simulink model "hysteresis_pam3_compare"  (R2022a)
settings: Solver=FixedStepDiscrete  StartTime=0  StopTime=simple_stop_time  FixedStep=simple_ts  RelTol=1e-3
undefined symbols (not defined in the file): simple_cfg, simple_ts
Description:
  | Structural preview, not MATLAB-saved or Simulink-tested. Run START_SIMULINK_COMPARE to rebuild natively and validate.
settings SolverCC: AlgebraicLoopSolver=TrustRegion
settings DataIOCC: SaveFormat=Array  SaveOutput=off  SignalLogging=off  TimeSaveName=simple_time
settings OptimizationCC: LifeSpan=inf
settings DebuggingCC: UnconnectedInputMsg=warning  UnconnectedOutputMsg=warning  UnconnectedLineMsg=warning  SFMachineParentedDataDiag=warning  ArithmeticOperatorsInVariantConditions=warning
settings SFSimCC: SimUseLocalCustomCode=off  CustomCodeUndefinedFunction=UseInterfaceOnly
settings RTWCC: RTWUseLocalCustomCode=off  DLArmComputeVersion=19.05
settings CodeAppCC: StateflowObjectComments=on

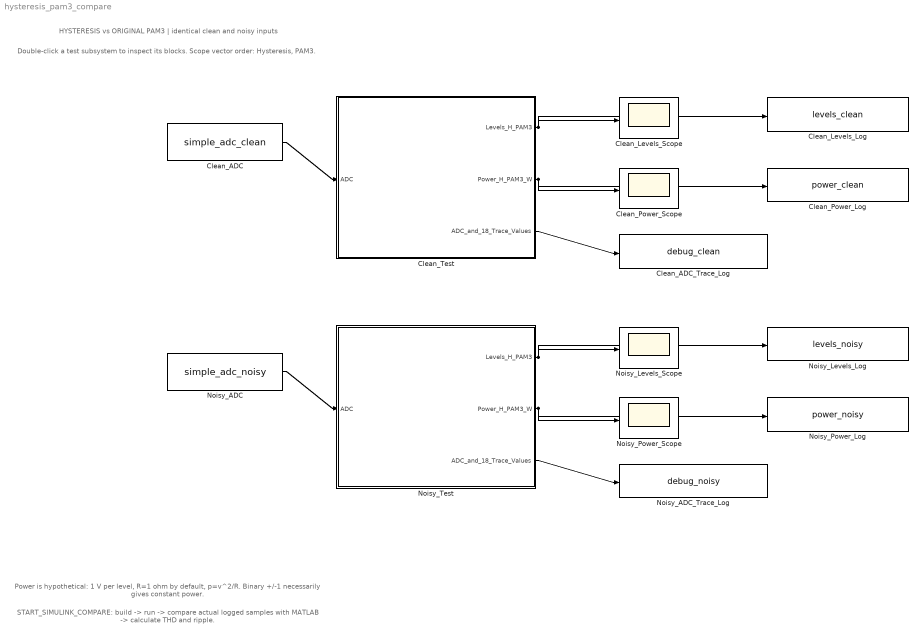
== system hysteresis_pam3_compare ==
  note: HYSTERESIS vs ORIGINAL PAM3 | identical clean and noisy inputs
  note: Double-click a test subsystem to inspect its blocks. Scope vector order: Hysteresis, PAM3.
  note: Power is hypothetical: 1 V per level, R=1 ohm by default, p=v^2/R. Binary +/-1 necessarily gives constant power.
  note: START_SIMULINK_COMPARE: build -> run -> compare actual logged samples with MATLAB -> calculate THD and ripple.
  Clean_ADC : FromWorkspace  VariableName=simple_adc_clean  Interpolate=off  SampleTime=simple_ts  OutputAfterFinalValue=Holding final value
  Clean_Test : Subsystem
  Clean_Levels_Scope : Scope
  Clean_Levels_Log : ToWorkspace  VariableName=levels_clean  SaveFormat=Array  SampleTime=-1
  Clean_Power_Scope : Scope
  Clean_Power_Log : ToWorkspace  VariableName=power_clean  SaveFormat=Array  SampleTime=-1
  Clean_ADC_Trace_Log : ToWorkspace  VariableName=debug_clean  SaveFormat=Array  SampleTime=-1
  Noisy_ADC : FromWorkspace  VariableName=simple_adc_noisy  Interpolate=off  SampleTime=simple_ts  OutputAfterFinalValue=Holding final value
  Noisy_Test : Subsystem
  Noisy_Levels_Scope : Scope
  Noisy_Levels_Log : ToWorkspace  VariableName=levels_noisy  SaveFormat=Array  SampleTime=-1
  Noisy_Power_Scope : Scope
  Noisy_Power_Log : ToWorkspace  VariableName=power_noisy  SaveFormat=Array  SampleTime=-1
  Noisy_ADC_Trace_Log : ToWorkspace  VariableName=debug_noisy  SaveFormat=Array  SampleTime=-1
  wires:
  Clean_ADC/1 -> Clean_Test/1(ADC)
  Clean_Test/1(Levels_H_PAM3) -> Clean_Levels_Scope/1, Clean_Levels_Log/1
  Clean_Test/2(Power_H_PAM3_W) -> Clean_Power_Scope/1, Clean_Power_Log/1
  Clean_Test/3(ADC_and_18_Trace_Values) -> Clean_ADC_Trace_Log/1
  Noisy_ADC/1 -> Noisy_Test/1(ADC)
  Noisy_Test/1(Levels_H_PAM3) -> Noisy_Levels_Scope/1, Noisy_Levels_Log/1
  Noisy_Test/2(Power_H_PAM3_W) -> Noisy_Power_Scope/1, Noisy_Power_Log/1
  Noisy_Test/3(ADC_and_18_Trace_Values) -> Noisy_ADC_Trace_Log/1

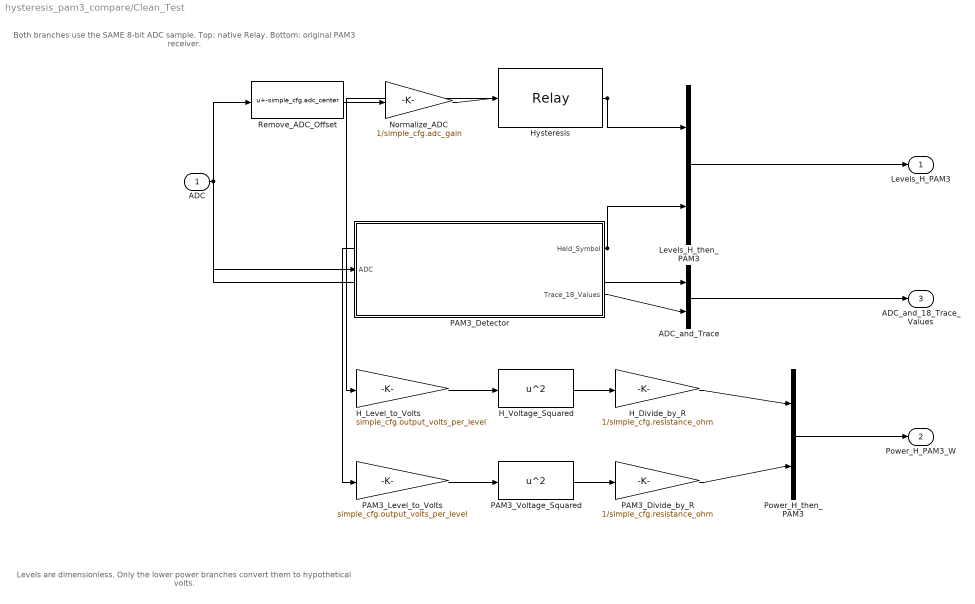
== system hysteresis_pam3_compare/Clean_Test ==
  note: Both branches use the SAME 8-bit ADC sample. Top: native Relay. Bottom: original PAM3 receiver.
  note: Levels are dimensionless. Only the lower power branches convert them to hypothetical volts.
  ADC : Inport  Port=1
  Remove_ADC_Offset : Bias  Bias=-simple_cfg.adc_center
  Normalize_ADC : Gain  Gain=1/simple_cfg.adc_gain
  Hysteresis : Relay  OnSwitchValue=simple_cfg.hysteresis_on  OffSwitchValue=simple_cfg.hysteresis_off  OnOutputValue=1  OffOutputValue=-1
  PAM3_Detector : Subsystem
  Levels_H_then_PAM3 : Mux  Inputs=2
  Levels_H_PAM3 : Outport  Port=1
  H_Level_to_Volts : Gain  Gain=simple_cfg.output_volts_per_level
  H_Voltage_Squared : Math  Operator=square
  H_Divide_by_R : Gain  Gain=1/simple_cfg.resistance_ohm
  PAM3_Level_to_Volts : Gain  Gain=simple_cfg.output_volts_per_level
  PAM3_Voltage_Squared : Math  Operator=square
  PAM3_Divide_by_R : Gain  Gain=1/simple_cfg.resistance_ohm
  Power_H_then_PAM3 : Mux  Inputs=2
  Power_H_PAM3_W : Outport  Port=2
  ADC_and_Trace : Mux  Inputs=2
  ADC_and_18_Trace_Values : Outport  Port=3
  wires:
  H_Level_to_Volts/1 -> H_Voltage_Squared/1
  H_Voltage_Squared/1 -> H_Divide_by_R/1
  PAM3_Level_to_Volts/1 -> PAM3_Voltage_Squared/1
  PAM3_Voltage_Squared/1 -> PAM3_Divide_by_R/1
  ADC/1 -> Remove_ADC_Offset/1, PAM3_Detector/1(ADC), ADC_and_Trace/1
  Remove_ADC_Offset/1 -> Normalize_ADC/1
  Normalize_ADC/1 -> Hysteresis/1
  Hysteresis/1 -> Levels_H_then_PAM3/1, H_Level_to_Volts/1
  PAM3_Detector/1(Held_Symbol) -> Levels_H_then_PAM3/2, PAM3_Level_to_Volts/1
  Levels_H_then_PAM3/1 -> Levels_H_PAM3/1
  H_Divide_by_R/1 -> Power_H_then_PAM3/1
  PAM3_Divide_by_R/1 -> Power_H_then_PAM3/2
  Power_H_then_PAM3/1 -> Power_H_PAM3_W/1
  PAM3_Detector/2(Trace_18_Values) -> ADC_and_Trace/2
  ADC_and_Trace/1 -> ADC_and_18_Trace_Values/1

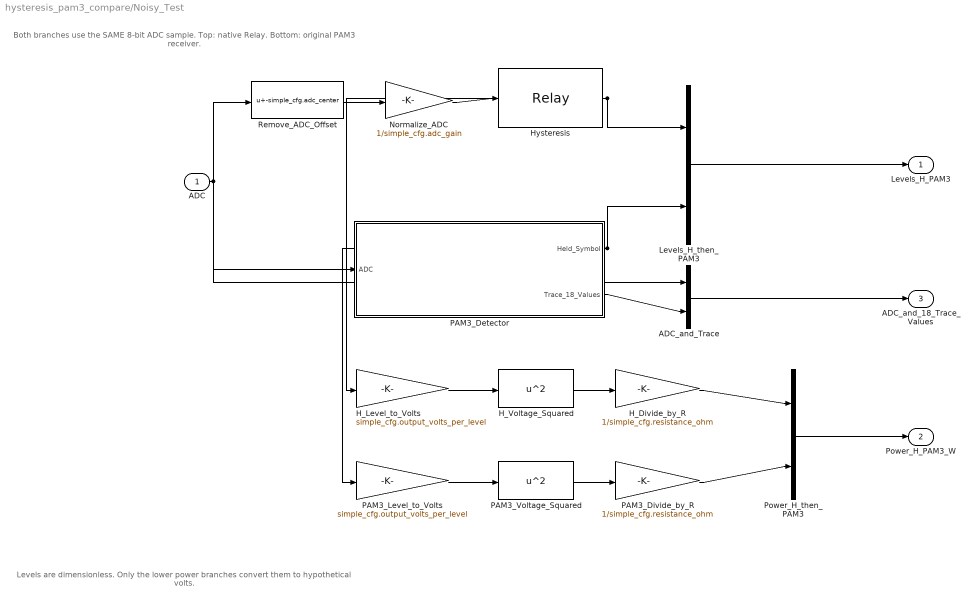
== system hysteresis_pam3_compare/Noisy_Test ==
  note: Both branches use the SAME 8-bit ADC sample. Top: native Relay. Bottom: original PAM3 receiver.
  note: Levels are dimensionless. Only the lower power branches convert them to hypothetical volts.
  ADC : Inport  Port=1
  Remove_ADC_Offset : Bias  Bias=-simple_cfg.adc_center
  Normalize_ADC : Gain  Gain=1/simple_cfg.adc_gain
  Hysteresis : Relay  OnSwitchValue=simple_cfg.hysteresis_on  OffSwitchValue=simple_cfg.hysteresis_off  OnOutputValue=1  OffOutputValue=-1
  PAM3_Detector : Subsystem
  Levels_H_then_PAM3 : Mux  Inputs=2
  Levels_H_PAM3 : Outport  Port=1
  H_Level_to_Volts : Gain  Gain=simple_cfg.output_volts_per_level
  H_Voltage_Squared : Math  Operator=square
  H_Divide_by_R : Gain  Gain=1/simple_cfg.resistance_ohm
  PAM3_Level_to_Volts : Gain  Gain=simple_cfg.output_volts_per_level
  PAM3_Voltage_Squared : Math  Operator=square
  PAM3_Divide_by_R : Gain  Gain=1/simple_cfg.resistance_ohm
  Power_H_then_PAM3 : Mux  Inputs=2
  Power_H_PAM3_W : Outport  Port=2
  ADC_and_Trace : Mux  Inputs=2
  ADC_and_18_Trace_Values : Outport  Port=3
  wires:
  H_Level_to_Volts/1 -> H_Voltage_Squared/1
  H_Voltage_Squared/1 -> H_Divide_by_R/1
  PAM3_Level_to_Volts/1 -> PAM3_Voltage_Squared/1
  PAM3_Voltage_Squared/1 -> PAM3_Divide_by_R/1
  ADC/1 -> Remove_ADC_Offset/1, PAM3_Detector/1(ADC), ADC_and_Trace/1
  Remove_ADC_Offset/1 -> Normalize_ADC/1
  Normalize_ADC/1 -> Hysteresis/1
  Hysteresis/1 -> Levels_H_then_PAM3/1, H_Level_to_Volts/1
  PAM3_Detector/1(Held_Symbol) -> Levels_H_then_PAM3/2, PAM3_Level_to_Volts/1
  Levels_H_then_PAM3/1 -> Levels_H_PAM3/1
  H_Divide_by_R/1 -> Power_H_then_PAM3/1
  PAM3_Divide_by_R/1 -> Power_H_then_PAM3/2
  Power_H_then_PAM3/1 -> Power_H_PAM3_W/1
  PAM3_Detector/2(Trace_18_Values) -> ADC_and_Trace/2
  ADC_and_Trace/1 -> ADC_and_18_Trace_Values/1

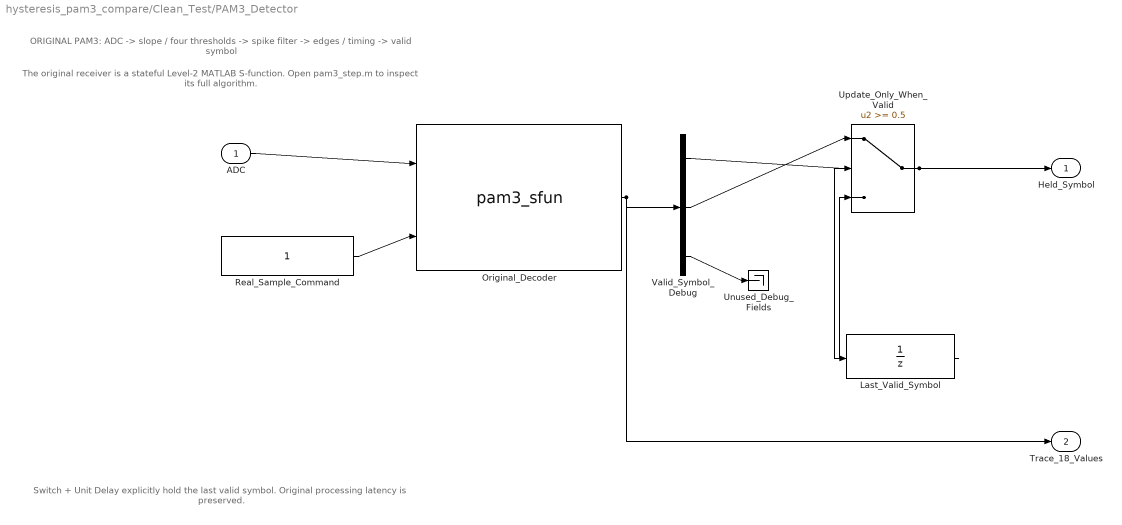
== system hysteresis_pam3_compare/Clean_Test/PAM3_Detector ==
  note: ORIGINAL PAM3: ADC -> slope / four thresholds -> spike filter -> edges / timing -> valid symbol
  note: The original receiver is a stateful Level-2 MATLAB S-function. Open pam3_step.m to inspect its full algorithm.
  note: Switch + Unit Delay explicitly hold the last valid symbol. Original processing latency is preserved.
  ADC : Inport  Port=1
  Real_Sample_Command : Constant  Value=1  SampleTime=simple_ts
  Original_Decoder : M-S-Function  FunctionName=pam3_sfun  Parameters=simple_pam3_cfg
  Valid_Symbol_Debug : Demux  Outputs=[1 1 16]
  Unused_Debug_Fields : Terminator
  Update_Only_When_Valid : Switch  Criteria=u2 >= Threshold  Threshold=0.5
  Last_Valid_Symbol : UnitDelay  InitialCondition=0  SampleTime=simple_ts
  Held_Symbol : Outport  Port=1
  Trace_18_Values : Outport  Port=2
  wires:
  ADC/1 -> Original_Decoder/1
  Real_Sample_Command/1 -> Original_Decoder/2
  Original_Decoder/1 -> Valid_Symbol_Debug/1, Trace_18_Values/1
  Valid_Symbol_Debug/2 -> Update_Only_When_Valid/1
  Valid_Symbol_Debug/1 -> Update_Only_When_Valid/2
  Valid_Symbol_Debug/3 -> Unused_Debug_Fields/1
  Last_Valid_Symbol/1 -> Update_Only_When_Valid/3
  Update_Only_When_Valid/1 -> Last_Valid_Symbol/1, Held_Symbol/1

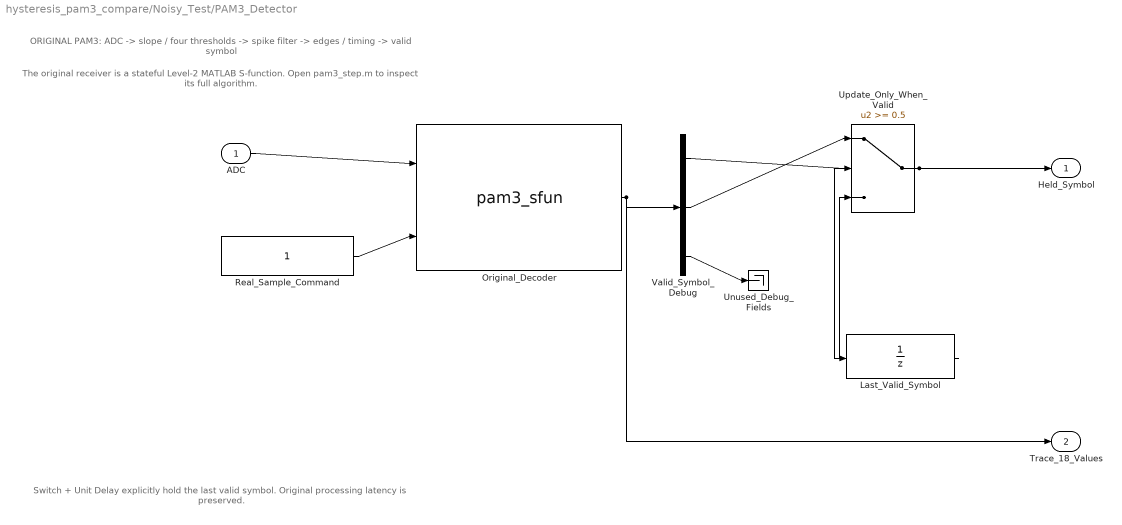
== system hysteresis_pam3_compare/Noisy_Test/PAM3_Detector ==
  note: ORIGINAL PAM3: ADC -> slope / four thresholds -> spike filter -> edges / timing -> valid symbol
  note: The original receiver is a stateful Level-2 MATLAB S-function. Open pam3_step.m to inspect its full algorithm.
  note: Switch + Unit Delay explicitly hold the last valid symbol. Original processing latency is preserved.
  ADC : Inport  Port=1
  Real_Sample_Command : Constant  Value=1  SampleTime=simple_ts
  Original_Decoder : M-S-Function  FunctionName=pam3_sfun  Parameters=simple_pam3_cfg
  Valid_Symbol_Debug : Demux  Outputs=[1 1 16]
  Unused_Debug_Fields : Terminator
  Update_Only_When_Valid : Switch  Criteria=u2 >= Threshold  Threshold=0.5
  Last_Valid_Symbol : UnitDelay  InitialCondition=0  SampleTime=simple_ts
  Held_Symbol : Outport  Port=1
  Trace_18_Values : Outport  Port=2
  wires:
  ADC/1 -> Original_Decoder/1
  Real_Sample_Command/1 -> Original_Decoder/2
  Original_Decoder/1 -> Valid_Symbol_Debug/1, Trace_18_Values/1
  Valid_Symbol_Debug/2 -> Update_Only_When_Valid/1
  Valid_Symbol_Debug/1 -> Update_Only_When_Valid/2
  Valid_Symbol_Debug/3 -> Unused_Debug_Fields/1
  Last_Valid_Symbol/1 -> Update_Only_When_Valid/3
  Update_Only_When_Valid/1 -> Last_Valid_Symbol/1, Held_Symbol/1
